simulink model "Stage4_PLL_STNF_K60"  (R2024b)
settings: Solver=ode1  StartTime=0.0  StopTime=2  FixedStep=Ts  RelTol=1e-3
InitFcn:
  | %% ===== Global =====
  | Ts = 1e-6;                        % pas d'echantillonnage [s]
  | 
  | %% ===== PV (module 550 W, rapport) =====
  | Nser = 14;  Npar = 4;
  | % Donnees du module : recopiees EN DUR dans le bloc PV Array
  | % (le masque n'accepte pas de variables dans Module data)
  | Ncell_mod = 144;
  | Voc_mod = 49.80;  Isc_mod = 13.98;
  | Vm_mod  = 41.95;  Im_mod  = 13.12;
  | kVoc = -0.270;    kIsc = 0.048;   % [%/deg.C]
  | C_pv = 470e-6;                    % condensateur PV [F]
  | 
  | %% ===== Profil d'eclairement =====
  | G1     = 1000;                    % [W/m2] avant l'echelon
  | G2     = 700;                     % [W/m2] apres l'echelon
  | t_step = 1;                       % [s] instant de l'echelon
  | 
  | %% ===== Boost PV =====
  | L_boost = 7.97e-3;                % [H]
  | C_dc    = 3e-3;                   % [F] condensateur du bus
  | fsw_dc  = 10e3;                   % [Hz]
  | D_test  = 0.344;                  % D fixe (etape 3.0, bloc commente)
  | R_dc    = 26;                     % [ohm] (etape 3.0, non utilise)
  | 
  | %% ===== MPPT IncCond =====
  | T_mppt = 20e-3;   % periode MPPT [s]
  | dD     = 0.005;                   % pas de perturbation
  | D0     = 0.25;                    % > 1 - Voc/V_ref = 0.23
  | D_min  = 0.05;
  | D_max  = 0.9;
  | 
  | %% ===== Filtre anti-repliement des mesures MPPT =====
  | tau_f = 0.5e-3;                   % [s]
  | a_f   = exp(-Ts/tau_f);
  | 
  | %% ===== Bus DC fixe (etape 3, retire a l'etape 4.3) =====
  | V_bus = 900;                      % [V]
  | R_bus = 0.1;                      % [ohm]
  | 
  | %% ===== Batterie (Etape 4) =====
  | V_bat_nom = 196;                  % [V] tension nominale NiMH
  | Q_bat     = 150;                  % [Ah] capacite
  | SOC0      = 80;                   % [%] etat de charge initial
  | 
  | %% ===== Hacheur bidirectionnel =====
  | L_bat     = 3e-3;                 % [H] redimensionnee (au lieu de 5 H)
  | fsw_bat   = 10e3;                 % [Hz]
  | I_bat_max = 30;                   % [A] saturation de la reference
  | 
  | %% ===== Boucle de courant (interne) : fc ~ 1 kHz =====
  | Kp_i = 0.021;                     % = wc*L_bat/V_ref
  | Ki_i = 26;                        % zero a wc/5
  | 
  | %% ===== Boucle de tension du bus (externe) : fc ~ 50 Hz =====
  | V_ref = 900;                      % [V]
  | Kp_v  = 4.3;                      % = wc*C_dc/(1-D), D = 1 - V_bat/V_ref
  | Ki_v  = 270;                      % zero a wc/5
  | 
  | %% ===== Charge DC =====
  | R_load = 30;                      % [ohm] ~ 27 kW a 900 V
  | %% ===== Test boucle de courant (etape 4.2) =====
  | I_ref1  = 20;                  % [A] decharge
  | I_ref2  = -20;                 % [A] charge
  | t_iref  = 1.5;                 % [s] instant de l'inversion
  | D0_bat  = 1 - 213/V_bus;       % D initial (Vbat a vide ~213 V)
  | Dbat_min = 0.05;
  | Dbat_max = 0.95;
  | %% ===== Etape 4.3 : bus regule par la batterie =====
  | Voc_array = Nser*Voc_mod;
  | D0        = 1 - 0.85*Voc_array/V_ref;
  | Vpv0      = Voc_array;
  | R_load    = 40.5;    % [ohm] charge permanente ~20 kW
  | %% ===== Etape 4.5 : delestage de charge =====
  | R_load2 = 133;                          % [ohm] charge delestable ~6.1 kW
  | t_load  = 1.5;                          % [s] instant du delestage
  | %% ===== Etape 4.6 : rampe de temperature =====
  | T1   = 25;       % [degC] temperature initiale
  | T2   = 45;       % [degC] temperature finale
  | t_T1 = 2;        % [s] debut de la rampe
  | t_T2 = 2.8;      % [s] fin de la rampe
  | %% ===== Etape 5 : onduleur triphase (boucle ouverte) =====
  | f_grid  = 50;                          % [Hz] frequence du reseau (Algerie)
  | V_ph    = 230;                         % [V rms] tension simple visee
  | m_inv   = V_ph*2*sqrt(2)/V_ref;        % indice de modulation (SPWM) ~0.72
  | fsw_inv = 10e3;                        % [Hz] frequence de decoupage onduleur
  | L_f     = 5e-3;                        % [H] inductance de filtre (par phase)
  | C_f     = 15e-6;                       % [F] capacite de filtre (par phase)
  | P_ac    = 26e3;                        % [W] puissance de la charge AC
  | R_ac    = 3*V_ph^2/P_ac;               % [ohm] charge par phase (etoile) ~6.1
  | V_LL = sqrt(3)*V_ph;                   % [V rms] tension composee ~400 V
  | Q_Cf = 3*V_ph^2*2*pi*f_grid*C_f;       % [var] puissance reactive de C_f ~747 var
  | %% ===== Etape 5.3 : compensation de la chute dans L_f =====
  | k_Lf  = abs(1 + 1j*2*pi*f_grid*L_f*(1/R_ac + 1j*2*pi*f_grid*C_f));  % ~1.026
  | m_inv = k_Lf*V_ph*2*sqrt(2)/V_ref;                                   % ~0.741
  | %% ===== Etape 6a : PLL SRF =====
  | Vm     = sqrt(2)*V_ph;      % amplitude de la tension simple [V]
  | w0     = 2*pi*f_grid;       % pulsation nominale [rad/s]
  | fn_pll = 20;  zeta = 0.707;  wn = 2*pi*fn_pll;
  | Kp_pll = 2*zeta*wn/Vm;      % ~0,55
  | Ki_pll = wn^2/Vm;           % ~48,6
  | dw_max = 2*pi*5;            % saturation du PI : +/- 5 Hz
  | %% ===== Etape 6b : raccordement au reseau =====
  | S_cc     = 1e6;      % puissance de court-circuit du reseau [VA]
  | XR_grid  = 7;        % rapport X/R du reseau
  | %% ===== Etape 6b : boucle de courant de l'onduleur =====
  | L_g    = (V_LL^2/S_cc)*XR_grid/sqrt(1+XR_grid^2)/(2*pi*f_grid);  % inductance du reseau [H]
  | L_tot  = L_f + L_g;               % inductance vue par la boucle de courant [H]
  | fc_i   = 500;                     % bande passante de la boucle de courant [Hz]
  | wc_i   = 2*pi*fc_i;
  | Kp_id  = wc_i*L_tot;              % ~17
  | Ki_id  = Kp_id*wc_i/5;            % ~10 900
  | P_ref  = 7e3;                     % puissance injectee : batterie dans ses limites (+/- 6,4 kW) a 400 et 100 W/m2                   % puissance active injectee au reseau [W]
  | Id_ref = 2*P_ref/(3*Vm);          % consigne de courant d'axe d [A], ~20,5
  | Q_ref = 0;                        % puissance reactive demandee [var] (0 -> cos phi = 1)
  | %% ===== SMC base sur le modele =====
  | % --- Onduleur (axes d et q) ---
  | R_tot  = (V_LL^2/S_cc)/sqrt(1+XR_grid^2);  % resistance du reseau ~0,023 ohm
  | A_port = 722;                               % amplitude de la porteuse MLI
  | k_MLI  = A_port/(V_ref/2);                  % 722/450 = 1,604
  | K1_st  = 40/L_tot;
  | K2_st  = 20000/L_tot;
  | tau_ff = 2e-3;              % filtre de l'anticipation (2 ms)
  | a_ff   = exp(-Ts/tau_ff);
  | % --- Batterie (courant) ---
  | R_b    = 0.023;                             % resistance interne batterie [ohm]
  | K1_bat = 14000;                             % gain K1 boucle courant batterie
  | K2_bat = 4e7;                               % gain K2 boucle courant batterie
  | % --- Bus DC (tension) ---
  | K1_v   = 3500;                              % gain K1 boucle tension bus (1400 x 2,5)
  | K2_v   = 5e5;                               % gain K2 boucle tension bus (2e5 x 2,5)
  | phi_v  = 0.5;                               % couche limite ST_v [V] : sign(S) -> sat(S/phi_v)
  | a_pf = exp(-Ts/1e-3);   % filtre 1 ms pour P_pv
  | 
  | %% ===== PLL Super-Twisting (document pll_sta_complet.pdf) =====
  | k1_pll = 30;                      % gain k1 (rad/s)
  | k2_pll = 150;                     % gain k2 (rad/s^2)
  | %% ===== Perturbation du reseau (echelon d'impedance) =====
  | t_p   = 0.75;                     % instant de la perturbation [s] (mettre 100 pour la supprimer)
  | SCR_p = 5;                        % SCR apres la perturbation (avant : 100)
  | XR_p  = 7;                        % rapport X/R apres la perturbation
  | Z_p   = V_LL^2/(SCR_p*10e3);      % impedance du reseau faible [ohm]
  | dR_p  = max(Z_p/sqrt(1+XR_p^2) - R_tot, 1e-9);                       % resistance ajoutee [ohm]
  | dL_p  = max(Z_p*XR_p/sqrt(1+XR_p^2)/(2*pi*f_grid) - L_g, 1e-9);      % inductance ajoutee [H]
  | 
  | %% ===== PLL Super-Twisting + N_F (dernier reglage) =====
  | k1_pll    = 60;     % gain proportionnel (rad/s)
  | k2_pll    = 600;    % gain integral (rad/s^2)
  | eps_pll   = 12;     % borne de la barriere (degres)
  | beta_pll  = 3;      % puissance en haut
  | gamma_pll = 3;      % puissance en bas
  | Nmax_pll  = 3;      % saturation de N_F (zone prouvee)
  | %% ===== Perturbation de frequence du reseau =====
  | df_reseau = 5;      % saut de frequence (Hz) : +5 ou -5 (0 = pas de perturbation)
  | t_f       = 0.75;   % instant du saut (s)
  | t_p       = 100;    % (ancienne perturbation d'impedance : desactivee)
undefined symbols (not defined in the file or in its folder): DiscIntNeverNeededParam, dspblkCoreblockFVToolHelper, gcbh, Hydride, Metal, Nickel, sgn
libraries: slpidlib x5, spsSeriesRLCBranchLib x3, spsVoltageMeasurementLib x3, spsUniversalBridgeLib x2, spsPWMGeneratorDCDCLib x2, spsabctodq0Lib x2, spsCurrentMeasurementLib x2, spsThreePhaseSeriesRLCBranchLib x2, spsBatteryLib x1, spsParallelRLCBranchLib x1, spsdq0toabcLib x1, spsPVArrayLib x1
(part 1 of 2)
settings Model: Creator=WINDOWS  LastModifiedBy=WINDOWS

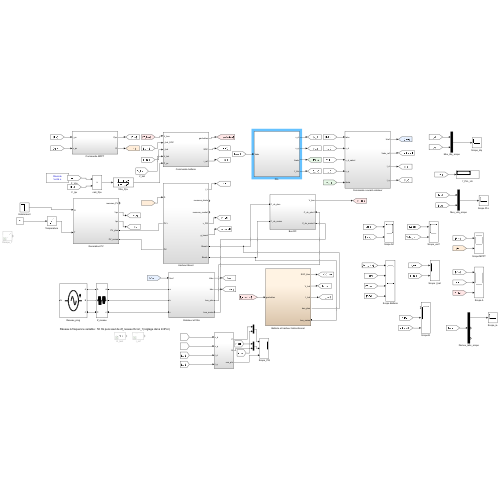
[thumbnail: Simulink's stored preview of the top-level diagram]
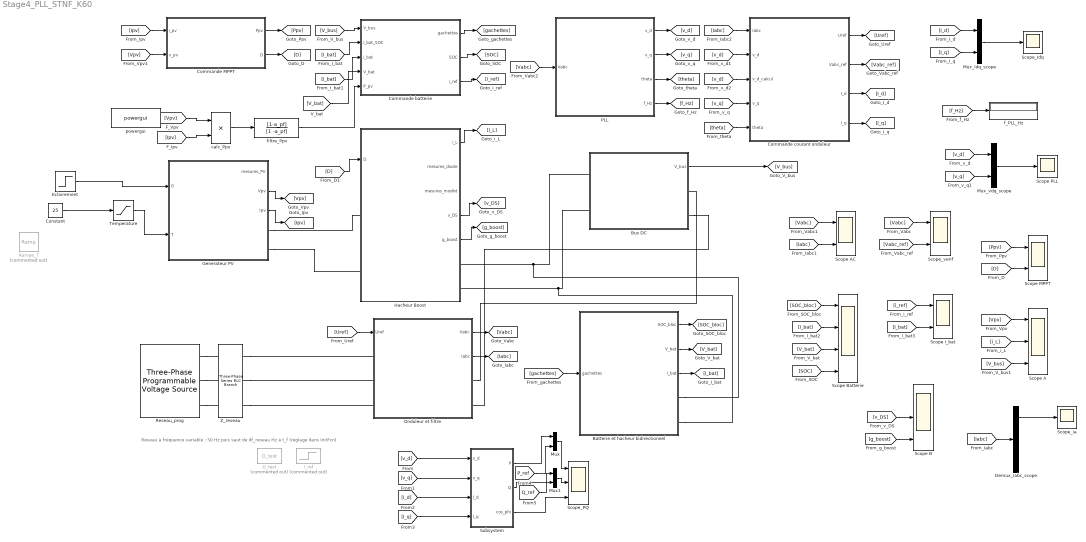
== system Stage4_PLL_STNF_K60 ==
  note: Réseau à fréquence variable : 50 Hz puis saut de df_reseau Hz à t_f (réglage dans InitFcn)
  Batterie et hacheur bidirectionnel : Subsystem
  Bus DC : Subsystem
  Commande MPPT : Subsystem
  Commande batterie : Subsystem
  Commande courant onduleur : Subsystem
  Constant : Constant  Value=25
  D_test : Constant  Commented=on  Value=D_test
  Demux_Iabc_scope : Demux  Outputs=3
  Eclairement : Step  Before=1000  After=200  SampleTime=Ts
  Generateur PV : Subsystem
  Hacheur Boost : Subsystem
  I_ref : Step  Commented=on  Time=t_iref  Before=I_ref1  After=I_ref2  SampleTime=Ts
  Mux : Mux  Inputs=2
  Mux1 : Mux  Inputs=2
  Mux_Idq_scope : Mux  Inputs=2
  Mux_vdq_scope : Mux  Inputs=2
  Onduleur et filtre : Subsystem
  PLL : Subsystem
  Rampe_T : simulink/Sources/Ramp  Commented=on  slope=(T2-T1)/(t_T2-t_T1)  start=t_T1  InitialOutput=T1
  Reseau_prog : spsThreePhaseProgrammableVoltageSourceLib/Three-Phase Programmable Voltage Source  PositiveSequence=[V_LL 0 50]  VariationEntity=Frequency  VariationType=Table of time-amplitude pairs  VariationTypeAlt=Step  VariationStep=df_reseau  VariationRate=10  VariationMagnitude=0.3  VariationFrequency=2  VariationTiming=[t_f 100]  VariationPhaseA=off  Amplitudes=[1 0.8 1.2 1.0]  TimeValues=[0 0.1 0.15 0.2]  HarmonicGeneration=off  HarmonicA=[3 0.2 -25 0]  HarmonicB=[2 0.15 35 2]  Timing="[0.05  3]"  BusType=swing  Pref=0  Qref=0  Qmin=-inf  Qmax=inf
  Scope A : Scope  NumInputPorts=3
  Scope AC : Scope  NumInputPorts=2
  Scope B : Scope  NumInputPorts=3
  Scope Batterie : Scope  NumInputPorts=4
  Scope I_bat : Scope  NumInputPorts=2
  Scope MPPT : Scope  NumInputPorts=2
  Scope PLL : Scope
  Scope_Idq : Scope
  Scope_PQ : Scope  NumInputPorts=3
  Scope_ia : Scope
  Scope_verif : Scope  NumInputPorts=2
  Subsystem : Subsystem
  Temperature : Saturate  UpperLimit=T2  LowerLimit=T1
  Z_reseau : spsThreePhaseSeriesRLCBranchLib/Three-Phase Series RLC Branch  LConnTagsString=A|B|C  RConnTagsString=A|B|C  BranchType=RL  Resistance=R_tot  Inductance=L_g  Capacitance=1e-6  Measurements=None
  calc_Ppv : Product
  f_PLL_Hz : Display
  filtre_Ppv : DiscreteTransferFcn  Numerator=[1-a_pf]  Denominator=[1 -a_pf]  SampleTime=Ts
  powergui : spspowerguiLib/powergui  Priority=1  SimulationMode=Discrete  SampleTime=1e-06  frequency=60  Iterations=50  frequencyindice=0  Pbase=100e6  ErrMax=1e-4  UnitsV=kV  UnitsW=MW  buscounter=0  FunctionMessages=off  echomessages=off  EnableUseOfTLC=off  CurrentSourceSwitches=off  DisableSnubberDevices=off  DisableRonSwitches=off  DisableVfSwitches=off  DisplayEquations=off  AutomaticDiscreteSolvers=off  SolverType=Tustin/Backward Euler (TBE)  Interpol=off  ExternalGateDelay=off  methode=off  Ts=100  x0status=blocks  SPID=on  SwTol=0  HookPort=off  NonlinearTolerance=1e-4  nMaxIteration=100  ContinueOnMaxIteration=off  RestoreLinks=warning  ResistiveCurrentMeasurement=off  Frange=[0:2:500]  Ylog=off  Xlog=on  ShowGrid=off  save=off  variable=ZData  structure=0  ZoomFFT=off  StartTime=0.0  cycles=1  DisplayStyle=1  fundamental=60  FreqAxis=off  MaxFrequency=1000  frequencyindicesteady=1  RmsSteady=1  display=off
  wires:
  Mux_vdq_scope/1 -> Scope PLL/1
  Demux_Iabc_scope/1 -> Scope_ia/1
  Mux_Idq_scope/1 -> Scope_Idq/1
  Hacheur Boost/5(g_boost) -> [g_boost]
  [g_boost] -> Scope B/3
  Hacheur Boost/4(v_DS) -> [v_DS]
  [v_DS] -> Scope B/2
  Hacheur Boost/1(i_L) -> [i_L]
  [i_L] -> Scope A/2
  Bus DC/1(V_bus) -> [V_bus]
  [V_bus] -> Commande batterie/1(V_bus)
  [V_bus] -> Scope A/3
  Commande MPPT/2(D) -> [D]
  [D] -> Scope MPPT/2
  [D] -> Hacheur Boost/1(D)
  Commande courant onduleur/4(I_q) -> [I_q]
  [I_q] -> Mux_Idq_scope/2
  Commande courant onduleur/3(I_d) -> [I_d]
  [I_d] -> Mux_Idq_scope/1
  Commande courant onduleur/2(Vabc_ref) -> [Vabc_ref]
  [Vabc_ref] -> Scope_verif/2
  Commande courant onduleur/1(Uref) -> [Uref]
  [Uref] -> Onduleur et filtre/1(Uref)
  Generateur PV/2(Vpv) -> [Vpv]
  [Vpv] -> Scope A/1
  [Vpv] -> Commande MPPT/2(v_pv)
  Commande MPPT/1(Ppv) -> [Ppv]
  [Ppv] -> Scope MPPT/1
  Onduleur et filtre/2(Iabc) -> [Iabc]
  [Iabc] -> Demux_Iabc_scope/1
  [Iabc] -> Scope AC/2
  [Iabc] -> Commande courant onduleur/1(Iabc)
  Onduleur et filtre/1(Vabc) -> [Vabc]
  [Vabc] -> Scope_verif/1
  [Vabc] -> Scope AC/1
  [Vabc] -> PLL/1(Vabc)
  Commande batterie/3(i_ref) -> [i_ref]
  [i_ref] -> Scope I_bat/1
  Commande batterie/2(SOC) -> [SOC]
  [SOC] -> Scope Batterie/4
  Commande batterie/1(gachettes) -> [gachettes]
  [gachettes] -> Batterie et hacheur bidirectionnel/1(gachettes)
  Batterie et hacheur bidirectionnel/1(SOC_bloc) -> [SOC_bloc]
  [SOC_bloc] -> Scope Batterie/1
  Batterie et hacheur bidirectionnel/3(I_bat) -> [I_bat]
  [I_bat] -> Commande batterie/2(i_bat_SOC)
  [I_bat] -> Commande batterie/3(i_bat)
  [I_bat] -> Scope Batterie/2
  [I_bat] -> Scope I_bat/2
  PLL/1(v_d) -> [v_d]
  [v_d] -> Mux_vdq_scope/1
  [v_d] -> Commande courant onduleur/2(v_d)
  [v_d] -> Commande courant onduleur/3(v_d_calcul)
  PLL/2(v_q) -> [v_q]
  [v_q] -> Commande courant onduleur/4(v_q)
  [v_q] -> Mux_vdq_scope/2
  PLL/3(theta) -> [theta]
  [theta] -> Commande courant onduleur/5(theta)
  PLL/4(f_Hz) -> [f_Hz]
  [f_Hz] -> f_PLL_Hz/1
  Batterie et hacheur bidirectionnel/2(V_bat) -> [V_bat]
  [V_bat] -> Scope Batterie/3
  Generateur PV/3(Ipv) -> [Ipv]
  [Ipv] -> Commande MPPT/1(i_pv)
  Temperature/1 -> Generateur PV/2(T)
  Constant/1 -> Temperature/1
  Eclairement/1 -> Generateur PV/1(G)
  [v_d] -> Subsystem/1(v_d)
  [v_q] -> Subsystem/2(v_q)
  [I_d] -> Subsystem/3(I_d)
  [I_q] -> Subsystem/4(I_q)
  Subsystem/3(cos_phi) -> Scope_PQ/3
  Subsystem/1(P) -> Mux/1
  [P_ref] -> Mux/2
  Mux/1 -> Scope_PQ/1
  Subsystem/2(Q) -> Mux1/1
  [Q_ref] -> Mux1/2
  Mux1/1 -> Scope_PQ/2
  [V_bat] -> Commande batterie/4(V_bat)
  [Vpv] -> calc_Ppv/1
  [Ipv] -> calc_Ppv/2
  calc_Ppv/1 -> filtre_Ppv/1
  filtre_Ppv/1 -> Commande batterie/5(P_pv)
  connections:
  Generateur PV/RConn2 -- Hacheur Boost/LConn2
  Bus DC/LConn1 -- Batterie et hacheur bidirectionnel/RConn1 -- Hacheur Boost/RConn1
  Bus DC/LConn2 -- Batterie et hacheur bidirectionnel/RConn2 -- Hacheur Boost/RConn2
  Onduleur et filtre/RConn1 -- Bus DC/RConn1
  Bus DC/RConn2 -- Onduleur et filtre/RConn2
  Generateur PV/RConn1 -- Hacheur Boost/LConn1
  Reseau_prog/RConn1 -- Z_reseau/LConn1
  Z_reseau/RConn1 -- Onduleur et filtre/LConn1
  Reseau_prog/RConn2 -- Z_reseau/LConn2
  Z_reseau/RConn2 -- Onduleur et filtre/LConn2
  Reseau_prog/RConn3 -- Z_reseau/LConn3
  Z_reseau/RConn3 -- Onduleur et filtre/LConn3

== system Stage4_PLL_STNF_K60/Batterie et hacheur bidirectionnel ==
  gachettes : Inport
  Batterie : spsBatteryLib/Battery  BatType=Nickel-Metal-Hydride  NomV=350  NomQ=Q_bat  SOC=SOC0  Batt_Tr=3  PresetModel=on  MaxQ=161.5385  MinV=262.5  FullV=412.2881  Dis_rate=30  R=0.023333  Normal_OP=144.2308  expZone="[379.661            30]"
  Bras_bat : spsUniversalBridgeLib/Universal Bridge  Arms=1  SnubberResistance=1e5  SnubberCapacitance=inf  Device=MOSFET / Diodes  Ron=1e-3  Lon=0  ForwardVoltages="[  0  0  ]"  ForwardVoltage=0  GTOparameters=[ 10e-6 , 20e-6 ]  IGBTparameters=[ 1e-6 , 2e-6 ]  Measurements=None  Measurements_2=None  converterType=Rectifier
  L_bat : spsSeriesRLCBranchLib/Series RLC Branch  LConnTagsString=__new0  RConnTagsString=__new0  BranchType=L  Resistance=1  Inductance=L_bat  SetiL0=off  InitialCurrent=0  Capacitance=1e-6  Setx0=off  InitialVoltage=0  Measurements=None
  Mesures_batterie : BusSelector  OutputSignals=SOC (%),Current (A),Voltage (V)
  bus_plus : PMIOPort  Side=Right
  bus_moins : PMIOPort  Port=2  Side=Right
  SOC_bloc : Outport
  V_bat : Outport  Port=2
  I_bat : Outport  Port=3
  wires:
  Batterie/1 -> Mesures_batterie/1
  gachettes/1 -> Bras_bat/1
  Mesures_batterie/3 -> V_bat/1  "<Voltage (V)>"
  Mesures_batterie/2 -> I_bat/1  "<Current (A)>"
  Mesures_batterie/1 -> SOC_bloc/1  "<SOC (%)>"
  connections:
  Bras_bat/RConn1 -- bus_plus/RConn1
  Batterie/LConn1 -- L_bat/LConn1
  L_bat/RConn1 -- Bras_bat/LConn1
  Bras_bat/RConn2 -- Batterie/LConn2 -- bus_moins/RConn1

== system Stage4_PLL_STNF_K60/Bus DC ==
  C_dc : spsParallelRLCBranchLib/Parallel RLC Branch  LConnTagsString=a  RConnTagsString=__new0  BranchType=C  Resistance=1  Inductance=1e-3  SetiL0=off  InitialCurrent=0  Capacitance=C_dc  Setx0=on  InitialVoltage=V_ref  Measurements=None
  V_out : spsVoltageMeasurementLib/Voltage Measurement  PhasorSimulation=off  OutputType=Complex  PSBequivalent=0
  C_dc_plus : PMIOPort  Side=Left
  C_dc_moins : PMIOPort  Port=2  Side=Left
  C_dc_plus1 : PMIOPort  Port=3  Side=Right
  C_dc_moins1 : PMIOPort  Port=4  Side=Right
  V_bus : Outport
  wires:
  V_out/1 -> V_bus/1
  connections:
  C_dc_plus/RConn1 -- C_dc_plus1/RConn1 -- V_out/LConn1 -- C_dc/LConn1
  C_dc/RConn1 -- V_out/LConn2 -- C_dc_moins1/RConn1 -- C_dc_moins/RConn1

== system Stage4_PLL_STNF_K60/Commande MPPT ==
  i_pv : Inport
  v_pv : Inport  Port=2
  Filtre_I : DiscreteTransferFcn  LoadFcn=dspblkCoreblockFVToolHelper(gcbh,'load');  Numerator=[1-a_f]  Denominator=[1 -a_f]  InitialStates=Ts
      settings: CopyFcn=dspblkCoreblockFVToolHelper(gcbh,'copy');  DeleteFcn=dspblkCoreblockFVToolHelper(gcbh,'close');  ModelCloseFcn=dspblkCoreblockFVToolHelper(gcbh,'close');  PreSaveFcn=dspblkCoreblockFVToolHelper(gcbh,'presave');  PostSaveFcn=dspblkCoreblockFVToolHelper(gcbh,'postsave');  CloseFcn=dspblkCoreblockFVToolHelper(gcbh,'close');
  Filtre_V : DiscreteTransferFcn  LoadFcn=dspblkCoreblockFVToolHelper(gcbh,'load');  Numerator=[1-a_f]  Denominator=[1 -a_f]  InitialStates=Ts
      settings: CopyFcn=dspblkCoreblockFVToolHelper(gcbh,'copy');  DeleteFcn=dspblkCoreblockFVToolHelper(gcbh,'close');  ModelCloseFcn=dspblkCoreblockFVToolHelper(gcbh,'close');  PreSaveFcn=dspblkCoreblockFVToolHelper(gcbh,'presave');  PostSaveFcn=dspblkCoreblockFVToolHelper(gcbh,'postsave');  CloseFcn=dspblkCoreblockFVToolHelper(gcbh,'close');
  MPPT_IncCond : MATLAB Function  TreatAsAtomicUnit=on
  P_pv : Product
  ZOH_I : ZeroOrderHold  SampleTime=T_mppt
  ZOH_V : ZeroOrderHold  SampleTime=T_mppt
  Ppv : Outport
  D : Outport  Port=2
  wires:
  v_pv/1 -> Filtre_V/1
  i_pv/1 -> Filtre_I/1
  Filtre_V/1 -> ZOH_V/1
  Filtre_I/1 -> ZOH_I/1
  ZOH_V/1 -> P_pv/1, MPPT_IncCond/1(V)
  MPPT_IncCond/1(D) -> D/1
  ZOH_I/1 -> P_pv/2, MPPT_IncCond/2(I)
  P_pv/1 -> Ppv/1

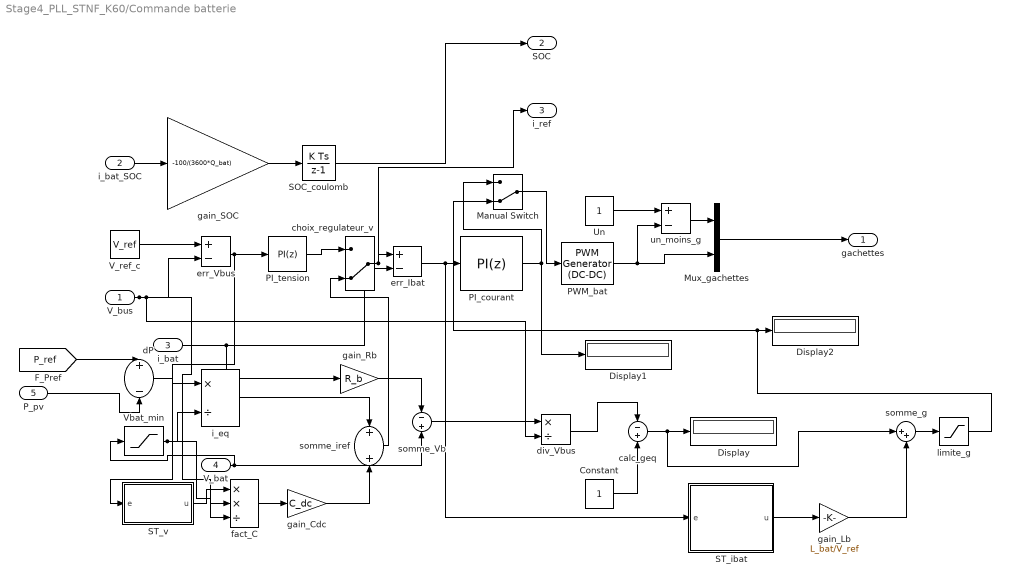
== system Stage4_PLL_STNF_K60/Commande batterie ==
  V_bus : Inport
  i_bat_SOC : Inport  Port=2
  i_bat : Inport  Port=3
  V_bat : Inport  Port=4
  P_pv : Inport  Port=5
  Constant : Constant
  Display : Display
  Display1 : Display
  Display2 : Display
  Manual Switch : ManualSwitch  CurrentSetting=0
  Mux_gachettes : Mux  Inputs=2
  PI_courant : slpidlib/PID Controller  Controller=PI  Form=Parallel  TimeDomain=Discrete-time  UseExternalTs=off  SampleTime=Ts  IntegratorMethod=Forward Euler  FilterMethod=Forward Euler  ControllerParametersSource=internal  P=Kp_i  I=Ki_i  UseKiTs=off  D=0  UseExternalDerivativeSource=off  N=100  UseFilter=on  TunerSelectOption=Transfer Function Based (PID Tuner App)  InitialConditionSource=internal  InitialConditionForIntegrator=D0_bat  InitialConditionForFilter=0  DifferentiatorICPrevScaledInput=0  ExternalReset=none  TrackingMode=off  Kt=1  LimitOutput=on  SatLimitsSource=internal  UpperSaturationLimit=Dbat_max  LowerSaturationLimit=Dbat_min  LinearizeAsGain=off  AntiWindupMode=clamping  Kb=1  LimitIntegrator=off  UpperIntegratorSaturationLimit=inf  LowerIntegratorSaturationLimit=-inf  POutMin=[]  POutMax=[]  IOutMin=[]  IOutMax=[]  DOutMin=[]  DOutMax=[]  NOutMin=[]  NOutMax=[]  SumOutMin=[]  SumOutMax=[]  SaturationOutMin=[]  SaturationOutMax=[]  PParamMin=[]  PParamMax=[]  IParamMin=[]  IParamMax=[]  DParamMin=[]  DParamMax=[]  NParamMin=[]  NParamMax=[]  KbParamMin=[]  KbParamMax=[]  KtParamMin=[]  KtParamMax=[]  KbOutMin=[]  KbOutMax=[]  KtOutMin=[]  KtOutMax=[]  IntegratorOutMin=[]  IntegratorOutMax=[]  FilterOutMin=[]  FilterOutMax=[]  SumI1OutMin=[]  SumI1OutMax=[]  SumI2OutMin=[]  SumI2OutMax=[]  SumI3OutMin=[]  SumI3OutMax=[]  SumI4OutMin=[]  SumI4OutMax=[]  SumDOutMin=[]  SumDOutMax=[]  DifferentiatorOutMin=[]  DifferentiatorOutMax=[]  FilterDiffOutCoefMin=[]  FilterDiffOutCoefMax=[]  ReciprocalOutMin=[]  ReciprocalOutMax=[]  SumDenOutMin=[]  SumDenOutMax=[]  SumNumOutMin=[]  SumNumOutMax=[]  DivideOutMin=[]  DivideOutMax=[]  UdiffTsProdOutMin=[]  UdiffTsProdOutMax=[]  NTsProdOutMin=[]  NTsProdOutMax=[]  UintegralTsProdOutMin=[]  UintegralTsProdOutMax=[]  UngainTsProdOutMin=[]  UngainTsProdOutMax=[]  ClampingZeroOutDataTypeStr=Inherit: Inherit via back propagation  ClampingZeroOutMin=[]  ClampingZeroOutMax=[]  FilterDenConstantOutDataTypeStr=Inherit: Inherit via back propagation  FilterDenConstantOutMin=[]  FilterDenConstantOutMax=[]  PCopyOutDataTypeStr=Inherit: Inherit via back propagation  PCopyOutMin=[]  PCopyOutMax=[]  NCopyOutDataTypeStr=Inherit: Inherit via back propagation  NCopyOutMin=[]  NCopyOutMax=[]  IntegratorContinuousStateAttributes=''  IntegratorStateMustResolveToSignalObject=off  IntegratorRTWStateStorageClass=Auto  FilterContinuousStateAttributes=''  FilterStateMustResolveToSignalObject=off  FilterRTWStateStorageClass=Auto  ParallelPVariant=InternalParameters  IdealPVariant=Disabled  IVariant=InternalParameters  DVariant=Disabled  IntegratorVariant=Discrete  SatVariant=Enabled  AWVariant=DiscClampingParallel  PCopyVariant=Disabled  TRVariant=Disabled  FdbkBlocksVariant=Forward  IdealPFdbkVariant=Disabled  SatFdbkVariant=Disabled  DerivativeFilterVariant=Disabled  NVariant=Disabled  NCopyVariant=Disabled_SignalSpec  FilterICVariant=Disabled  IntegratorICVariant=InternalICs  ExternalResetVariant=Disabled  TRSumVariant=Passthrough  SumFdbkVariant=Disabled  SumVariant=Sum_PI  TsampFilterVariant=InternalTs  TsampNgainVariant=Passthrough  TsampIntegralVariant=Disabled_SignalSpec  ExternalSaturationOutDataTypeStr=Inherit: Same as second input  DerivativeSourceVariant=Disabled  PreIntVariant=InternalPreInt
      settings: LibrarySourceBlock=simulink/Discrete/Discrete PID Controller
  PI_tension : slpidlib/PID Controller  Controller=PI  Form=Parallel  TimeDomain=Discrete-time  UseExternalTs=off  SampleTime=Ts  IntegratorMethod=Forward Euler  FilterMethod=Forward Euler  ControllerParametersSource=internal  P=Kp_v  I=Ki_v  UseKiTs=off  D=0  UseExternalDerivativeSource=off  N=100  UseFilter=on  TunerSelectOption=Transfer Function Based (PID Tuner App)  InitialConditionSource=internal  InitialConditionForIntegrator=0  InitialConditionForFilter=0  DifferentiatorICPrevScaledInput=0  ExternalReset=none  TrackingMode=off  Kt=1  LimitOutput=off  SatLimitsSource=internal  UpperSaturationLimit=I_bat_max  LowerSaturationLimit=-I_bat_max  LinearizeAsGain=off  AntiWindupMode=clamping  Kb=1  LimitIntegrator=off  UpperIntegratorSaturationLimit=inf  LowerIntegratorSaturationLimit=-inf  POutMin=[]  POutMax=[]  IOutMin=[]  IOutMax=[]  DOutMin=[]  DOutMax=[]  NOutMin=[]  NOutMax=[]  SumOutMin=[]  SumOutMax=[]  SaturationOutMin=[]  SaturationOutMax=[]  PParamMin=[]  PParamMax=[]  IParamMin=[]  IParamMax=[]  DParamMin=[]  DParamMax=[]  NParamMin=[]  NParamMax=[]  KbParamMin=[]  KbParamMax=[]  KtParamMin=[]  KtParamMax=[]  KbOutMin=[]  KbOutMax=[]  KtOutMin=[]  KtOutMax=[]  IntegratorOutMin=[]  IntegratorOutMax=[]  FilterOutMin=[]  FilterOutMax=[]  SumI1OutMin=[]  SumI1OutMax=[]  SumI2OutMin=[]  SumI2OutMax=[]  SumI3OutMin=[]  SumI3OutMax=[]  SumI4OutMin=[]  SumI4OutMax=[]  SumDOutMin=[]  SumDOutMax=[]  DifferentiatorOutMin=[]  DifferentiatorOutMax=[]  FilterDiffOutCoefMin=[]  FilterDiffOutCoefMax=[]  ReciprocalOutMin=[]  ReciprocalOutMax=[]  SumDenOutMin=[]  SumDenOutMax=[]  SumNumOutMin=[]  SumNumOutMax=[]  DivideOutMin=[]  DivideOutMax=[]  UdiffTsProdOutMin=[]  UdiffTsProdOutMax=[]  NTsProdOutMin=[]  NTsProdOutMax=[]  UintegralTsProdOutMin=[]  UintegralTsProdOutMax=[]  UngainTsProdOutMin=[]  UngainTsProdOutMax=[]  ClampingZeroOutDataTypeStr=Inherit: Inherit via back propagation  ClampingZeroOutMin=[]  ClampingZeroOutMax=[]  FilterDenConstantOutDataTypeStr=Inherit: Inherit via back propagation  FilterDenConstantOutMin=[]  FilterDenConstantOutMax=[]  PCopyOutDataTypeStr=Inherit: Inherit via back propagation  PCopyOutMin=[]  PCopyOutMax=[]  NCopyOutDataTypeStr=Inherit: Inherit via back propagation  NCopyOutMin=[]  NCopyOutMax=[]  IntegratorContinuousStateAttributes=''  IntegratorStateMustResolveToSignalObject=off  IntegratorRTWStateStorageClass=Auto  FilterContinuousStateAttributes=''  FilterStateMustResolveToSignalObject=off  FilterRTWStateStorageClass=Auto  ParallelPVariant=InternalParameters  IdealPVariant=Disabled  IVariant=InternalParameters  DVariant=Disabled  IntegratorVariant=Discrete  SatVariant=Disabled  AWVariant=Passthrough  PCopyVariant=Disabled  TRVariant=Disabled  FdbkBlocksVariant=Forward  IdealPFdbkVariant=Disabled  SatFdbkVariant=Disabled  DerivativeFilterVariant=Disabled  NVariant=Disabled  NCopyVariant=Disabled_SignalSpec  FilterICVariant=Disabled  IntegratorICVariant=InternalICs  ExternalResetVariant=Disabled  TRSumVariant=Passthrough  SumFdbkVariant=Disabled  SumVariant=Sum_PI  TsampFilterVariant=InternalTs  TsampNgainVariant=Passthrough  TsampIntegralVariant=Disabled_SignalSpec  ExternalSaturationOutDataTypeStr=Inherit: Same as second input  DerivativeSourceVariant=Disabled  PreIntVariant=InternalPreInt
      settings: LibrarySourceBlock=simulink/Discrete/Discrete PID Controller
  PWM_bat : spsPWMGeneratorDCDCLib/PWM Generator (DC-DC)  Fsw=fsw_bat  Ts=Ts
  SOC_coulomb : DiscreteIntegrator  SampleTime=-1  ICPrevOutput=DiscIntNeverNeededParam  ICPrevScaledInput=DiscIntNeverNeededParam
  ST_ibat : Subsystem
  ST_v : Subsystem
  Un : Constant
  V_ref_c : Constant  Value=V_ref
  Vbat_min : Saturate  UpperLimit=inf  LowerLimit=100
  calc_geq : Sum  Inputs=-+
  choix_regulateur_v : ManualSwitch  CurrentSetting=0
  dP : Sum  Inputs=+-
  div_Vbus : Product  Inputs=*/
  err_Ibat : Sum  Inputs=+-
  err_Vbus : Sum  Inputs=+-
  fact_C : Product  Inputs=**/
  gain_Cdc : Gain  Gain=C_dc
  gain_Lb : Gain  Gain=L_bat/V_ref
  gain_Rb : Gain  Gain=R_b
  gain_SOC : Gain  Gain=-100/(3600*Q_bat)
  i_eq : Product  Inputs=*/
  limite_g : Saturate  UpperLimit=Dbat_max  LowerLimit=Dbat_min
  somme_Vb : Sum  Inputs=-+
  somme_g : Sum  Inputs=|++
  somme_iref : Sum
  un_moins_g : Sum  Inputs=+-
  gachettes : Outport
  SOC : Outport  Port=2
  i_ref : Outport  Port=3
  wires:
  i_bat_SOC/1 -> gain_SOC/1
  SOC_coulomb/1 -> SOC/1
  V_ref_c/1 -> err_Vbus/1
  PI_courant/1 -> Display1/1, Manual Switch/1
  err_Vbus/1 -> PI_tension/1, ST_v/1(e)
  V_bus/1 -> div_Vbus/2, err_Vbus/2, fact_C/2
  gain_SOC/1 -> SOC_coulomb/1
  i_bat/1 -> gain_Rb/1, err_Ibat/2
  err_Ibat/1 -> ST_ibat/1(e), PI_courant/1
  Un/1 -> un_moins_g/1
  PWM_bat/1 -> Mux_gachettes/2, un_moins_g/2
  un_moins_g/1 -> Mux_gachettes/1
  Mux_gachettes/1 -> gachettes/1
  V_bat/1 -> somme_Vb/2, Vbat_min/1
  gain_Rb/1 -> somme_Vb/1
  somme_Vb/1 -> div_Vbus/1
  Constant/1 -> calc_geq/2
  div_Vbus/1 -> calc_geq/1
  calc_geq/1 -> somme_g/1, Display/1
  ST_ibat/1(u) -> gain_Lb/1
  gain_Lb/1 -> somme_g/2
  somme_g/1 -> limite_g/1
  limite_g/1 -> Manual Switch/2, Display2/1
  Manual Switch/1 -> PWM_bat/1
  [P_ref] -> dP/1
  P_pv/1 -> dP/2
  dP/1 -> i_eq/1
  Vbat_min/1 -> i_eq/2, fact_C/3
  ST_v/1(u) -> fact_C/1
  fact_C/1 -> gain_Cdc/1
  i_eq/1 -> somme_iref/1
  gain_Cdc/1 -> somme_iref/2
  PI_tension/1 -> choix_regulateur_v/1
  somme_iref/1 -> choix_regulateur_v/2
  choix_regulateur_v/1 -> i_ref/1, err_Ibat/1

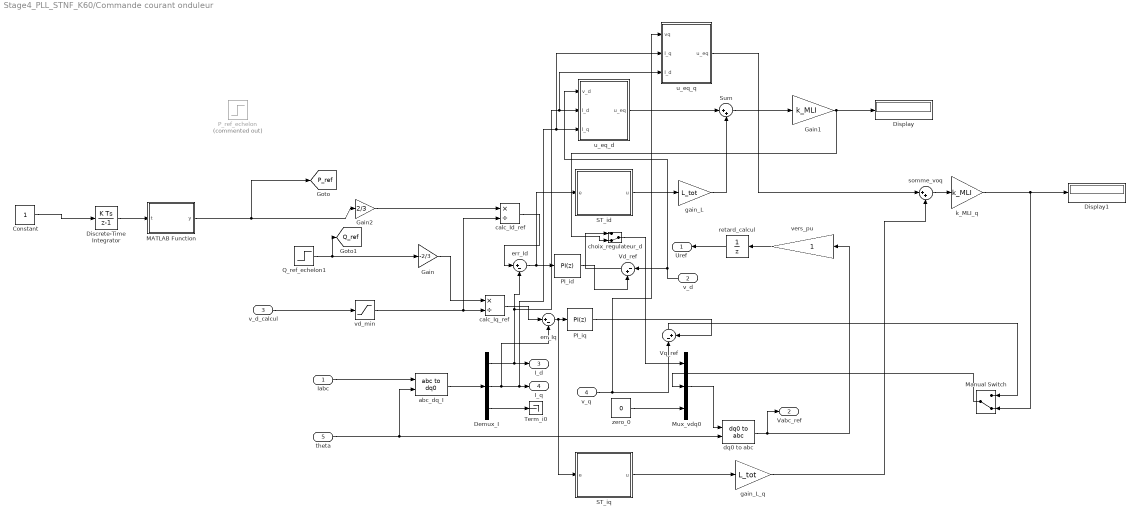
== system Stage4_PLL_STNF_K60/Commande courant onduleur ==
  Iabc : Inport
  v_d : Inport  Port=2
  v_d_calcul : Inport  Port=3
  v_q : Inport  Port=4
  theta : Inport  Port=5
  Constant : Constant
  Demux_I : Demux  Outputs=3
  Discrete-Time Integrator : DiscreteIntegrator  SampleTime=Ts  ICPrevOutput=DiscIntNeverNeededParam  ICPrevScaledInput=DiscIntNeverNeededParam
  Display : Display
  Display1 : Display
  Gain : Gain  Gain=-2/3
  Gain1 : Gain  Gain=k_MLI
  Gain2 : Gain  Gain=2/3
  MATLAB Function : MATLAB Function  TreatAsAtomicUnit=on
  Manual Switch : ManualSwitch  CurrentSetting=0
  Mux_vdq0 : Mux  Inputs=3
  PI_id : slpidlib/PID Controller  Controller=PI  Form=Parallel  TimeDomain=Discrete-time  UseExternalTs=off  SampleTime=Ts  IntegratorMethod=Forward Euler  FilterMethod=Forward Euler  ControllerParametersSource=internal  P=Kp_id  I=Ki_id  UseKiTs=off  D=0  UseExternalDerivativeSource=off  N=100  UseFilter=on  TunerSelectOption=Transfer Function Based (PID Tuner App)  InitialConditionSource=internal  InitialConditionForIntegrator=0  InitialConditionForFilter=0  DifferentiatorICPrevScaledInput=0  ExternalReset=none  TrackingMode=off  Kt=1  LimitOutput=off  SatLimitsSource=internal  UpperSaturationLimit=200  LowerSaturationLimit=-200  LinearizeAsGain=off  AntiWindupMode=clamping  Kb=1  LimitIntegrator=off  UpperIntegratorSaturationLimit=inf  LowerIntegratorSaturationLimit=-inf  POutMin=[]  POutMax=[]  IOutMin=[]  IOutMax=[]  DOutMin=[]  DOutMax=[]  NOutMin=[]  NOutMax=[]  SumOutMin=[]  SumOutMax=[]  SaturationOutMin=[]  SaturationOutMax=[]  PParamMin=[]  PParamMax=[]  IParamMin=[]  IParamMax=[]  DParamMin=[]  DParamMax=[]  NParamMin=[]  NParamMax=[]  KbParamMin=[]  KbParamMax=[]  KtParamMin=[]  KtParamMax=[]  KbOutMin=[]  KbOutMax=[]  KtOutMin=[]  KtOutMax=[]  IntegratorOutMin=[]  IntegratorOutMax=[]  FilterOutMin=[]  FilterOutMax=[]  SumI1OutMin=[]  SumI1OutMax=[]  SumI2OutMin=[]  SumI2OutMax=[]  SumI3OutMin=[]  SumI3OutMax=[]  SumI4OutMin=[]  SumI4OutMax=[]  SumDOutMin=[]  SumDOutMax=[]  DifferentiatorOutMin=[]  DifferentiatorOutMax=[]  FilterDiffOutCoefMin=[]  FilterDiffOutCoefMax=[]  ReciprocalOutMin=[]  ReciprocalOutMax=[]  SumDenOutMin=[]  SumDenOutMax=[]  SumNumOutMin=[]  SumNumOutMax=[]  DivideOutMin=[]  DivideOutMax=[]  UdiffTsProdOutMin=[]  UdiffTsProdOutMax=[]  NTsProdOutMin=[]  NTsProdOutMax=[]  UintegralTsProdOutMin=[]  UintegralTsProdOutMax=[]  UngainTsProdOutMin=[]  UngainTsProdOutMax=[]  ClampingZeroOutDataTypeStr=Inherit: Inherit via back propagation  ClampingZeroOutMin=[]  ClampingZeroOutMax=[]  FilterDenConstantOutDataTypeStr=Inherit: Inherit via back propagation  FilterDenConstantOutMin=[]  FilterDenConstantOutMax=[]  PCopyOutDataTypeStr=Inherit: Inherit via back propagation  PCopyOutMin=[]  PCopyOutMax=[]  NCopyOutDataTypeStr=Inherit: Inherit via back propagation  NCopyOutMin=[]  NCopyOutMax=[]  IntegratorContinuousStateAttributes=''  IntegratorStateMustResolveToSignalObject=off  IntegratorRTWStateStorageClass=Auto  FilterContinuousStateAttributes=''  FilterStateMustResolveToSignalObject=off  FilterRTWStateStorageClass=Auto  ParallelPVariant=InternalParameters  IdealPVariant=Disabled  IVariant=InternalParameters  DVariant=Disabled  IntegratorVariant=Discrete  SatVariant=Disabled  AWVariant=Passthrough  PCopyVariant=Disabled  TRVariant=Disabled  FdbkBlocksVariant=Forward  IdealPFdbkVariant=Disabled  SatFdbkVariant=Disabled  DerivativeFilterVariant=Disabled  NVariant=Disabled  NCopyVariant=Disabled_SignalSpec  FilterICVariant=Disabled  IntegratorICVariant=InternalICs  ExternalResetVariant=Disabled  TRSumVariant=Passthrough  SumFdbkVariant=Disabled  SumVariant=Sum_PI  TsampFilterVariant=InternalTs  TsampNgainVariant=Passthrough  TsampIntegralVariant=Disabled_SignalSpec  ExternalSaturationOutDataTypeStr=Inherit: Same as second input  DerivativeSourceVariant=Disabled  PreIntVariant=InternalPreInt
      settings: LibrarySourceBlock=simulink/Discrete/Discrete PID Controller
  PI_iq : slpidlib/PID Controller  Controller=PI  Form=Parallel  TimeDomain=Discrete-time  UseExternalTs=off  SampleTime=Ts  IntegratorMethod=Forward Euler  FilterMethod=Forward Euler  ControllerParametersSource=internal  P=Kp_id  I=Ki_id  UseKiTs=off  D=0  UseExternalDerivativeSource=off  N=100  UseFilter=on  TunerSelectOption=Transfer Function Based (PID Tuner App)  InitialConditionSource=internal  InitialConditionForIntegrator=0  InitialConditionForFilter=0  DifferentiatorICPrevScaledInput=0  ExternalReset=none  TrackingMode=off  Kt=1  LimitOutput=off  SatLimitsSource=internal  UpperSaturationLimit=200  LowerSaturationLimit=-200  LinearizeAsGain=off  AntiWindupMode=clamping  Kb=1  LimitIntegrator=off  UpperIntegratorSaturationLimit=inf  LowerIntegratorSaturationLimit=-inf  POutMin=[]  POutMax=[]  IOutMin=[]  IOutMax=[]  DOutMin=[]  DOutMax=[]  NOutMin=[]  NOutMax=[]  SumOutMin=[]  SumOutMax=[]  SaturationOutMin=[]  SaturationOutMax=[]  PParamMin=[]  PParamMax=[]  IParamMin=[]  IParamMax=[]  DParamMin=[]  DParamMax=[]  NParamMin=[]  NParamMax=[]  KbParamMin=[]  KbParamMax=[]  KtParamMin=[]  KtParamMax=[]  KbOutMin=[]  KbOutMax=[]  KtOutMin=[]  KtOutMax=[]  IntegratorOutMin=[]  IntegratorOutMax=[]  FilterOutMin=[]  FilterOutMax=[]  SumI1OutMin=[]  SumI1OutMax=[]  SumI2OutMin=[]  SumI2OutMax=[]  SumI3OutMin=[]  SumI3OutMax=[]  SumI4OutMin=[]  SumI4OutMax=[]  SumDOutMin=[]  SumDOutMax=[]  DifferentiatorOutMin=[]  DifferentiatorOutMax=[]  FilterDiffOutCoefMin=[]  FilterDiffOutCoefMax=[]  ReciprocalOutMin=[]  ReciprocalOutMax=[]  SumDenOutMin=[]  SumDenOutMax=[]  SumNumOutMin=[]  SumNumOutMax=[]  DivideOutMin=[]  DivideOutMax=[]  UdiffTsProdOutMin=[]  UdiffTsProdOutMax=[]  NTsProdOutMin=[]  NTsProdOutMax=[]  UintegralTsProdOutMin=[]  UintegralTsProdOutMax=[]  UngainTsProdOutMin=[]  UngainTsProdOutMax=[]  ClampingZeroOutDataTypeStr=Inherit: Inherit via back propagation  ClampingZeroOutMin=[]  ClampingZeroOutMax=[]  FilterDenConstantOutDataTypeStr=Inherit: Inherit via back propagation  FilterDenConstantOutMin=[]  FilterDenConstantOutMax=[]  PCopyOutDataTypeStr=Inherit: Inherit via back propagation  PCopyOutMin=[]  PCopyOutMax=[]  NCopyOutDataTypeStr=Inherit: Inherit via back propagation  NCopyOutMin=[]  NCopyOutMax=[]  IntegratorContinuousStateAttributes=''  IntegratorStateMustResolveToSignalObject=off  IntegratorRTWStateStorageClass=Auto  FilterContinuousStateAttributes=''  FilterStateMustResolveToSignalObject=off  FilterRTWStateStorageClass=Auto  ParallelPVariant=InternalParameters  IdealPVariant=Disabled  IVariant=InternalParameters  DVariant=Disabled  IntegratorVariant=Discrete  SatVariant=Disabled  AWVariant=Passthrough  PCopyVariant=Disabled  TRVariant=Disabled  FdbkBlocksVariant=Forward  IdealPFdbkVariant=Disabled  SatFdbkVariant=Disabled  DerivativeFilterVariant=Disabled  NVariant=Disabled  NCopyVariant=Disabled_SignalSpec  FilterICVariant=Disabled  IntegratorICVariant=InternalICs  ExternalResetVariant=Disabled  TRSumVariant=Passthrough  SumFdbkVariant=Disabled  SumVariant=Sum_PI  TsampFilterVariant=InternalTs  TsampNgainVariant=Passthrough  TsampIntegralVariant=Disabled_SignalSpec  ExternalSaturationOutDataTypeStr=Inherit: Same as second input  DerivativeSourceVariant=Disabled  PreIntVariant=InternalPreInt
      settings: LibrarySourceBlock=simulink/Discrete/Discrete PID Controller
  P_ref_echelon : Step  Commented=on  Before=8000  After=8000  SampleTime=0
  Q_ref_echelon1 : Step  Time=0.5  After=0  SampleTime=0
  ST_id : Subsystem
  ST_iq : Subsystem
  Sum : Sum  Inputs=|++
  Term_i0 : Terminator
  Vd_ref : Sum  Inputs=|-+
  Vq_ref : Sum  Inputs=|-+
  abc_dq_I : spsabctodq0Lib/abc to dq0  Alignment=90 degrees behind phase A axis
  calc_Id_ref : Product  Inputs=*/
  calc_Iq_ref : Product  Inputs=*/
  choix_regulateur_d : ManualSwitch  CurrentSetting=0
  dq0 to abc : spsdq0toabcLib/dq0 to abc  Alignment=90 degrees behind phase A axis
  err_Id : Sum  Inputs=|+-
  err_Iq : Sum  Inputs=|+-
  gain_L : Gain  Gain=L_tot
  gain_L_q : Gain  Gain=L_tot
  k_MLI_q : Gain  Gain=k_MLI
  retard_calcul : UnitDelay  SampleTime=Ts  HasFrameUpgradeWarning=on
  somme_voq : Sum  Inputs=|++
  u_eq_d : Subsystem
  u_eq_q : Subsystem
  vd_min : Saturate  UpperLimit=inf  LowerLimit=100
  vers_pu : Gain
  zero_0 : Constant  Value=0
  Uref : Outport
  Vabc_ref : Outport  Port=2
  I_d : Outport  Port=3
  I_q : Outport  Port=4
  tag scope: P_ref=global, Q_ref=global
  wires:
  Gain/1 -> calc_Iq_ref/1
  v_d/1 -> u_eq_d/1(v_d), Vd_ref/1
  Gain2/1 -> calc_Id_ref/1
  v_d_calcul/1 -> vd_min/1
  Iabc/1 -> abc_dq_I/1
  Q_ref_echelon1/1 -> [Q_ref], Gain/1
  theta/1 -> abc_dq_I/2, dq0 to abc/2
  vd_min/1 -> calc_Id_ref/2, calc_Iq_ref/2
  retard_calcul/1 -> Uref/1
  err_Id/1 -> ST_id/1(e), PI_id/1
  abc_dq_I/1 -> Demux_I/1
  calc_Iq_ref/1 -> err_Iq/1
  calc_Id_ref/1 -> err_Id/1
  Demux_I/1 -> err_Id/2, u_eq_q/3(I_d), u_eq_d/2(I_d), I_d/1
  v_q/1 -> u_eq_q/1(vq), Vq_ref/1
  Demux_I/2 -> err_Iq/2, u_eq_q/2(I_q), u_eq_d/3(I_q), I_q/1
  Demux_I/3 -> Term_i0/1
  err_Iq/1 -> ST_iq/1(e), PI_iq/1
  zero_0/1 -> Mux_vdq0/3
  Mux_vdq0/1 -> dq0 to abc/1
  dq0 to abc/1 -> vers_pu/1, Vabc_ref/1
  vers_pu/1 -> retard_calcul/1
  ST_id/1(u) -> gain_L/1
  ST_iq/1(u) -> gain_L_q/1
  u_eq_d/1(u_eq) -> Sum/1
  gain_L/1 -> Sum/2
  Sum/1 -> Gain1/1
  Gain1/1 -> choix_regulateur_d/2, Display/1
  PI_id/1 -> Vd_ref/2
  Vd_ref/1 -> choix_regulateur_d/1
  choix_regulateur_d/1 -> Mux_vdq0/1
  u_eq_q/1(u_eq) -> somme_voq/1
  gain_L_q/1 -> somme_voq/2
  somme_voq/1 -> k_MLI_q/1
  k_MLI_q/1 -> Display1/1, Manual Switch/2
  PI_iq/1 -> Vq_ref/2
  Vq_ref/1 -> Manual Switch/1
  Manual Switch/1 -> Mux_vdq0/2
  Constant/1 -> Discrete-Time Integrator/1
  Discrete-Time Integrator/1 -> MATLAB Function/1(t)
  MATLAB Function/1(y) -> Gain2/1, [P_ref]

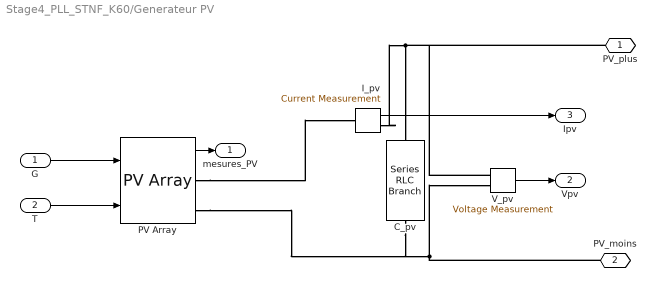
== system Stage4_PLL_STNF_K60/Generateur PV ==
  G : Inport
  T : Inport  Port=2
  C_pv : spsSeriesRLCBranchLib/Series RLC Branch  LConnTagsString=__new0  RConnTagsString=__new0  BranchType=C  Resistance=1  Inductance=1e-3  SetiL0=off  InitialCurrent=0  Capacitance=C_pv  Setx0=on  InitialVoltage=Vpv0  Measurements=None
  I_pv : spsCurrentMeasurementLib/Current Measurement  PhasorSimulation=off  OutputType=Complex  PSBequivalent=0
  PV Array : spsPVArrayLib/PV Array  Npar=04  Nser=14  PlotType=array @ 1000 W/m2 & specified temperatures  S_vec="[ 1000  500  100 ]"  Temp_C_vec="[50 45 25  ]"  ModuleName=User-defined  PlotWhenSelected=off  Pm=550.384  Ncell=144  Voc=49.80  Isc=13.98  Vm=41.95  Im=13.12  beta_Voc_pc=-0.270  alpha_Isc_pc=0.048  beta_Voc=-0.13446  alpha_Isc=0.0067104  IL=14.0374  I0=1.2644e-11  nI=0.48582  Rsh=125.1227  Rs=0.16535  RobustModel=off  RobustCellTemperature=313.3991  BAL=on  Tc=1e-6  Tfilter=5e-5
  V_pv : spsVoltageMeasurementLib/Voltage Measurement  PhasorSimulation=off  OutputType=Complex  PSBequivalent=0
  PV_plus : PMIOPort  Side=Right
  PV_moins : PMIOPort  Port=2  Side=Right
  mesures_PV : Outport
  Vpv : Outport  Port=2
  Ipv : Outport  Port=3
  wires:
  T/1 -> PV Array/2
  I_pv/1 -> Ipv/1
  G/1 -> PV Array/1
  V_pv/1 -> Vpv/1
  PV Array/1 -> mesures_PV/1
  connections:
  PV Array/RConn1 -- I_pv/LConn1
  PV_plus/RConn1 -- V_pv/LConn1 -- I_pv/RConn1 -- C_pv/LConn1
  PV_moins/RConn1 -- V_pv/LConn2 -- PV Array/RConn2 -- C_pv/RConn1

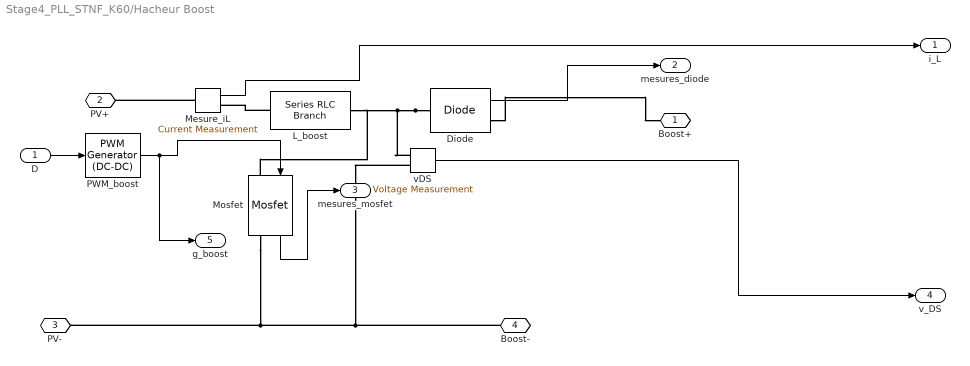
== system Stage4_PLL_STNF_K60/Hacheur Boost ==
  D : Inport
  Diode : spsDiodeLib/Diode  Ron=0.001  Lon=0  Vf=0.8  IC=0  UseSnubber=0  Rs=500  Cs=250e-9  Measurements=on
  L_boost : spsSeriesRLCBranchLib/Series RLC Branch  LConnTagsString=__new0  RConnTagsString=__new0  BranchType=L  Resistance=1  Inductance=L_boost  SetiL0=off  InitialCurrent=0  Capacitance=1e-6  Setx0=off  InitialVoltage=0  Measurements=None
  Mesure_iL : spsCurrentMeasurementLib/Current Measurement  PhasorSimulation=off  OutputType=Complex  PSBequivalent=0
  Mosfet : spsMosfetLib/Mosfet  Ron=0.1  Lon=0  Rd=0.01  Vfd=0  IC=0  Rs=1e5  Cs=inf  Measurements=on
  PWM_boost : spsPWMGeneratorDCDCLib/PWM Generator (DC-DC)  Fsw=fsw_dc  Ts=Ts
  vDS : spsVoltageMeasurementLib/Voltage Measurement  PhasorSimulation=off  OutputType=Complex  PSBequivalent=0
  Boost+ : PMIOPort  Side=Right
  PV+ : PMIOPort  Port=2  Side=Left
  PV- : PMIOPort  Port=3  Side=Left
  Boost- : PMIOPort  Port=4  Side=Right
  i_L : Outport
  mesures_diode : Outport  Port=2
  mesures_mosfet : Outport  Port=3
  v_DS : Outport  Port=4
  g_boost : Outport  Port=5
  wires:
  vDS/1 -> v_DS/1
  PWM_boost/1 -> g_boost/1, Mosfet/1
  Mesure_iL/1 -> i_L/1
  Diode/1 -> mesures_diode/1
  Mosfet/1 -> mesures_mosfet/1
  D/1 -> PWM_boost/1
  connections:
  L_boost/LConn1 -- Mesure_iL/RConn1
  Diode/LConn1 -- L_boost/RConn1 -- Mosfet/LConn1 -- vDS/LConn1
  vDS/LConn2 -- Boost-/RConn1 -- Mosfet/RConn1 -- PV-/RConn1
  Mesure_iL/LConn1 -- PV+/RConn1
  Diode/RConn1 -- Boost+/RConn1

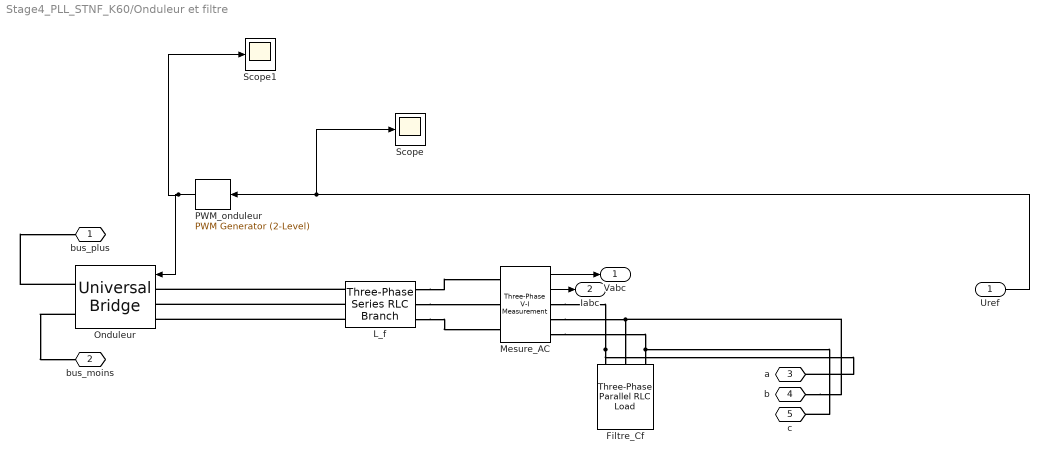
== system Stage4_PLL_STNF_K60/Onduleur et filtre ==
  Uref : Inport
  Filtre_Cf : spsThreePhaseParallelRLCLoadLib/Three-Phase Parallel RLC Load  LConnTagsString=A|B|C  Configuration=Y (grounded)  NominalVoltage=V_LL  Vabc=[1e3 1e3 1e3]  Vabcp=[1e3 1e3 1e3]  NominalFrequency=f_grid  UnbalancedPower=off  ActivePower=0  InductivePower=0  CapacitivePower=Q_Cf  Pabc=[10e3 9e3 11e3]  QLabc=[100 90 110]  QCabc=[100 90 110]  Pabcp=[10e3 9e3 11e3]  QLabcp=[100 90 110]  QCabcp=[100 90 110]  Measurements=None  LoadType=constant Z
  L_f : spsThreePhaseSeriesRLCBranchLib/Three-Phase Series RLC Branch  LConnTagsString=A|B|C  RConnTagsString=A|B|C  BranchType=L  Resistance=1  Inductance=L_f  Capacitance=1e-6  Measurements=None
  Mesure_AC : spsThreePhaseVIMeasurementLib/Three-Phase V-I Measurement  VoltageMeasurement=phase-to-ground  SetLabelV=off  LabelV=Vabc  Vpu=off  VpuLL=off  CurrentMeasurement=yes  SetLabelI=off  LabelI=Iabc  Ipu=off  Pbase=100e6  Vbase=500e3  OutputType=Complex  PhasorSimulation=off  PSBequivalent=0
  Onduleur : spsUniversalBridgeLib/Universal Bridge  Arms=3  SnubberResistance=1e5  SnubberCapacitance=inf  Device=IGBT / Diodes  Ron=1e-3  Lon=0  ForwardVoltages=[1.5 1.5]  ForwardVoltage=0  GTOparameters=[ 10e-6 , 20e-6 ]  IGBTparameters=[ 1e-6 , 2e-6 ]  Measurements=None  Measurements_2=None  converterType=Rectifier
  PWM_onduleur : spsPWMGenerator2LevelLib/PWM Generator (2-Level)  ModulatorType=Three-phase bridge (6 pulses)  ModulatorMode=Unsynchronized  Fc=fsw_inv  Pc=90  nF=27  MinMax="[ -722  722 ]"  SamplingTechnique=Natural  ModulatingSignals=off  m=m_inv  Freq=f_grid  Phase=0  Ts=Ts  ShowCarrierOutport=off
  Scope : Scope
  Scope1 : Scope
  bus_plus : PMIOPort  Side=Right
  bus_moins : PMIOPort  Port=2  Side=Right
  a : PMIOPort  Port=3  Side=Left
  b : PMIOPort  Port=4  Side=Left
  c : PMIOPort  Port=5  Side=Left
  Vabc : Outport
  Iabc : Outport  Port=2
  wires:
  PWM_onduleur/1 -> Scope1/1, Onduleur/1
  Mesure_AC/1 -> Vabc/1
  Uref/1 -> Scope/1, PWM_onduleur/1
  Mesure_AC/2 -> Iabc/1
  connections:
  L_f/RConn2 -- Mesure_AC/LConn2
  Mesure_AC/RConn1 -- a/RConn1 -- Filtre_Cf/LConn1
  Mesure_AC/RConn3 -- c/RConn1 -- Filtre_Cf/LConn3
  Mesure_AC/RConn2 -- b/RConn1 -- Filtre_Cf/LConn2
  Onduleur/RConn1 -- bus_plus/RConn1
  L_f/RConn1 -- Mesure_AC/LConn1
  L_f/RConn3 -- Mesure_AC/LConn3
  L_f/LConn3 -- Onduleur/LConn3
  L_f/LConn1 -- Onduleur/LConn1
  L_f/LConn2 -- Onduleur/LConn2
  Onduleur/RConn2 -- bus_moins/RConn1
